simulink model "structure_hifi"  (R2026b)
settings: Solver=VariableStepAuto
undefined symbols (not defined in the file or in its folder): DiscIntNeverNeededParam, P, Ts
settings Model: Creator=aomar  LastModifiedBy=aomar

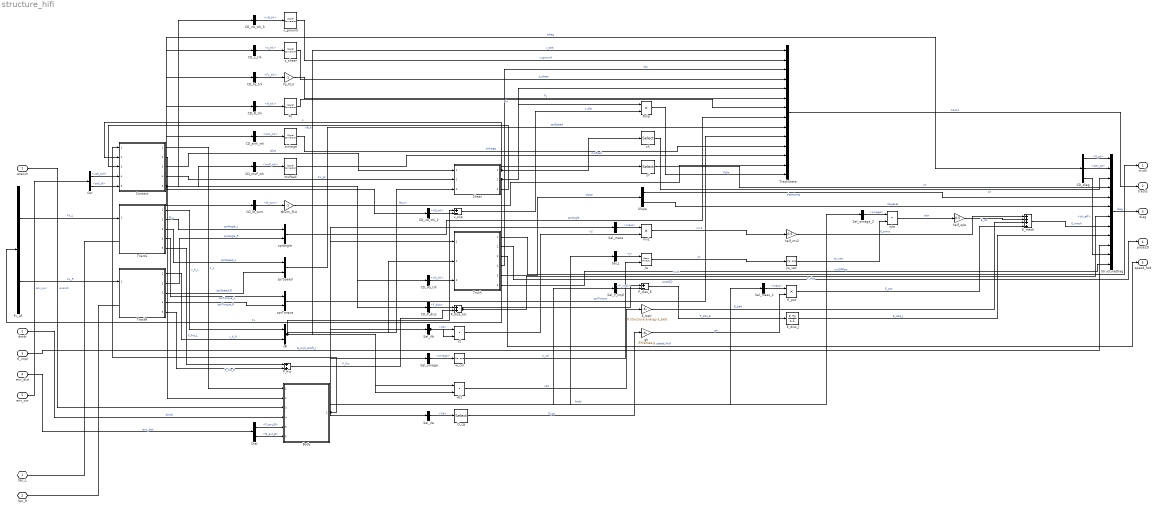
== system structure_hifi ==
  wrench : Inport
  dmdt : Inport  Port=2
  E_impl : Inport  Port=3
  env_dist : Inport  Port=4  OutDataTypeStr=Bus: Bus_EnvDisturbance
  env_ovr : Inport  Port=5  OutDataTypeStr=Bus: Bus_EnvOverride
  Body : Subsystem  ReferencedSubsystem=structure_body6dof
  CD_Fy_trk : BusSelector  OutputSignals=Fy_trk
  CD_M_turn : BusSelector  OutputSignals=M_turn
  CD_N_trk : BusSelector  OutputSignals=N_trk
  CD_P_diss : BusSelector  OutputSignals=P_diss
  CD_diag : BusSelector  OutputSignals=N_pt,pen_pt,chi_eff
  CD_muP_trk : BusSelector  OutputSignals=muP_trk
  CD_s_trk : BusSelector  OutputSignals=s_trk
  CD_sink_trk : BusSelector  OutputSignals=sink_trk
  CD_vG_trk : BusSelector  OutputSignals=vG_trk
  CD_vG_trk_2 : BusSelector  OutputSignals=vG_trk
  CD_vG_trk_3 : BusSelector  OutputSignals=vG_trk
  Contact : Subsystem  ReferencedSubsystem=structure_contact
  D_cg : Selector  InputPortWidth=3  IndexOptions=Index vector (dialog)  Indices=3  OutputSizes=1
  Dist : BusSelector  OutputSignals=F_ext_B,M_ext_B
  E_belt : Gain  Gain=P.structure.energy.k_belt
  E_diss_J : DiscreteIntegrator  gainval=1  SampleTime=Ts.base  ICPrevOutput=DiscIntNeverNeededParam  ICPrevScaledInput=DiscIntNeverNeededParam
  E_mech : Sum  Inputs=++++
  E_pot : Product  Inputs=**
  Fn : SignalConversion  OverrideOpt=off
  Fx_LR : Demux  Outputs=2
  Fy_FLU : Gain  Gain=-1
  Jw : Product  Inputs=**  Multiplication=Matrix(*)
  Jw_vec : Reshape
  Mturn_FLU : Gain  Gain=-1
  Ovr : BusSelector  OutputSignals=use_soil,soil_id
  P_diss_E : Sum  Inputs=+-
  P_diss_tot : Sum
  P_fric : Sum
  Pslip : Product  Inputs=**
  Sel_J : BusSelector  OutputSignals=J
  Sel_P_impl : BusSelector  OutputSignals=P_impl
  Sel_Vb : BusSelector  OutputSignals=Vb
  Sel_Xe : BusSelector  OutputSignals=Xe
  Sel_mass : BusSelector  OutputSignals=mass
  Sel_mass_2 : BusSelector  OutputSignals=mass
  Sel_omega : BusSelector  OutputSignals=omega
  Sel_omega_2 : BusSelector  OutputSignals=omega
  Shear : Subsystem  ReferencedSubsystem=structure_track_shear
  Slope : Demux  Outputs=2
  StructureDiag : BusCreator  Inputs=12  OutDataTypeStr=Bus: Bus_StructureDiag  NonVirtualBus=on
  TrackL : Subsystem  ReferencedSubsystem=structure_track_side  side=1 left
  TrackR : Subsystem  ReferencedSubsystem=structure_track_side  side=2 right
  TrackState : BusCreator  Inputs=14  OutDataTypeStr=Bus: Bus_TrackState  NonVirtualBus=on
  Truth : Subsystem  ReferencedSubsystem=structure_truth
  gh : Gain  Gain=-P.frames.g
  half_mv2 : Gain  Gain=0.5
  half_wJw : Gain  Gain=0.5
  muPeak : SignalConversion  OverrideOpt=off
  mv2 : Product  Inputs=**
  sX : Selector  InputPortWidth=4*P.structure.track.Nc  IndexOptions=Index vector (dialog)  Indices=1:2*P.structure.track.Nc  OutputSizes=1
  sY : Selector  InputPortWidth=4*P.structure.track.Nc  IndexOptions=Index vector (dialog)  Indices=2*P.structure.track.Nc+1:4*P.structure.track.Nc  OutputSizes=1
  s_shear : SignalConversion  OverrideOpt=off
  sinkage : SignalConversion  OverrideOpt=off
  sprAngle : Mux  Inputs=2
  sprSpeed : Mux  Inputs=2
  sprTorque : Mux  Inputs=2
  v2 : DotProduct  OutDataTypeStr=Inherit: Inherit via internal rule
  vB : Mux  Inputs=2
  v_ground : SignalConversion  OverrideOpt=off
  v_slip : Sum  Inputs=+-
  vb2 : DotProduct  OutDataTypeStr=Inherit: Inherit via internal rule
  wJw : DotProduct  OutDataTypeStr=Inherit: Inherit via internal rule
  w_col : Reshape  OutputDimensionality=Column vector (2-D)
  Spr_L : PMIOPort  Side=Left  ConnectionType=Connection: foundation.mechanical.rotational.rotational
  Spr_R : PMIOPort  Port=2  Side=Left  ConnectionType=Connection: foundation.mechanical.rotational.rotational
  truth : Outport  OutDataTypeStr=Bus: Bus_TruthState
  tracks : Outport  Port=2  OutDataTypeStr=Bus: Bus_TrackState
  diag : Outport  Port=3  OutDataTypeStr=Bus: Bus_StructureDiag
  pose2D : Outport  Port=4
  speed_fwd : Outport  Port=5
  wires:
  Fx_LR/1 -> TrackL/1  "Fx_L"
  Fx_LR/2 -> TrackR/1  "Fx_R"
  wrench/1 -> Body/3  "wrench"
  dmdt/1 -> Body/4  "dmdt"
  E_impl/1 -> StructureDiag/10  "E_impl_shaft_J"
  env_dist/1 -> Dist/1  "env_dist"
  env_ovr/1 -> Ovr/1  "env_ovr"
  Ovr/1 -> Contact/4  "<use_soil>"
  Ovr/2 -> Contact/5  "<soil_id>"
  Contact/1 -> Body/1  "F_c"
  Contact/2 -> Body/2  "M_c"
  Contact/3 -> Shear/1  "sDot"
  Contact/4 -> Shear/2  "Fx_pt"
  Contact/5 -> CD_vG_trk_3/1, CD_s_trk/1, CD_P_diss/1, CD_Fy_trk/1, CD_vG_trk/1, CD_N_trk/1, CD_sink_trk/1, CD_vG_trk_2/1, CD_muP_trk/1, CD_M_turn/1, CD_diag/1  "cdiag"
  TrackL/1 -> vB/1  "v_b_L"
  TrackL/2 -> sprAngle/1  "sprAngle_L"
  TrackL/3 -> sprSpeed/1  "sprSpeed_L"
  TrackL/4 -> sprTorque/1  "sprTorque_L"
  TrackL/5 -> P_fric/1  "P_fric_L"
  TrackR/1 -> vB/2  "v_b_R"
  TrackR/2 -> sprAngle/2  "sprAngle_R"
  TrackR/3 -> sprSpeed/2  "sprSpeed_R"
  TrackR/4 -> sprTorque/2  "sprTorque_R"
  TrackR/5 -> P_fric/2  "P_fric_R"
  CD_vG_trk_3/1 -> v_ground/1  "<vG_trk>"
  CD_s_trk/1 -> s_shear/1  "<s_trk>"
  CD_Fy_trk/1 -> Fy_FLU/1  "<Fy_trk>"
  CD_N_trk/1 -> Fn/1  "<N_trk>"
  CD_sink_trk/1 -> sinkage/1  "<sink_trk>"
  CD_muP_trk/1 -> muPeak/1  "<muP_trk>"
  CD_M_turn/1 -> Mturn_FLU/1  "<M_turn>"
  Dist/1 -> Body/5  "<F_ext_B>"
  Dist/2 -> Body/6  "<M_ext_B>"
  sprAngle/1 -> TrackState/8  "sprAngle"
  sprSpeed/1 -> TrackState/9  "sprSpeed"
  sprTorque/1 -> TrackState/10  "sprTorque"
  vB/1 -> TrackState/1, Shear/3, v_slip/1, Truth/2, vb2/2, vb2/1  "v_belt"
  P_fric/1 -> P_diss_tot/2  "P_fric"
  Fy_FLU/1 -> TrackState/6  "Fy"
  Mturn_FLU/1 -> TrackState/13  "Mturn"
  v_ground/1 -> TrackState/2  "v_ground"
  s_shear/1 -> TrackState/4  "s_shear"
  Fn/1 -> TrackState/7  "Fn"
  sinkage/1 -> TrackState/11  "sinkage"
  muPeak/1 -> TrackState/12  "muPeak"
  Body/1 -> Contact/1, Sel_omega_2/1, Sel_mass/1, Truth/1, Sel_J/1, Sel_P_impl/1, Sel_mass_2/1, Sel_Vb/1, Sel_omega/1, Sel_Xe/1  "body"
  CD_vG_trk_2/1 -> v_slip/2  "<vG_trk>"
  CD_vG_trk/1 -> Truth/3  "<vG_trk>"
  CD_P_diss/1 -> P_diss_tot/1  "<P_diss>"
  Sel_Vb/1 -> v2/2, v2/1  "<Vb>"
  Sel_omega/1 -> w_col/1  "<omega>"
  Sel_Xe/1 -> D_cg/1  "<Xe>"
  v_slip/1 -> Pslip/2  "v_slip"
  P_diss_tot/1 -> StructureDiag/7, P_diss_E/1  "P_diss"
  v2/1 -> mv2/2  "v2"
  w_col/1 -> Jw/2  "w_col"
  vb2/1 -> E_belt/1  "vb2"
  D_cg/1 -> gh/1  "D_cg"
  Shear/1 -> sX/1, Contact/2, sY/1  "s"
  Shear/2 -> TrackState/5, Pslip/1, Fx_LR/1  "Fx"
  Shear/3 -> Contact/3  "vB_d"
  Truth/1 -> truth/1  "truth"
  Truth/2 -> pose2D/1  "pose2D"
  Truth/3 -> speed_fwd/1  "speed_fwd"
  Truth/4 -> TrackState/3  "slip"
  Truth/5 -> Slope/1  "slope"
  Truth/6 -> StructureDiag/12  "outOfMap"
  Sel_mass/1 -> mv2/1  "<mass>"
  Sel_J/1 -> Jw/1  "<J>"
  Sel_P_impl/1 -> P_diss_E/2  "<P_impl>"
  Slope/1 -> StructureDiag/5  "slopeLong"
  Slope/2 -> StructureDiag/6  "slopeLat"
  P_diss_E/1 -> E_diss_J/1  "P_diss_E"
  Pslip/1 -> TrackState/14  "Pslip"
  mv2/1 -> half_mv2/1  "mv2"
  Jw/1 -> Jw_vec/1  "Jw"
  E_belt/1 -> E_mech/3  "E_belt"
  gh/1 -> E_pot/2  "gh"
  sX/1 -> StructureDiag/3  "sX"
  sY/1 -> StructureDiag/4  "sY"
  Sel_mass_2/1 -> E_pot/1  "<mass>"
  TrackState/1 -> tracks/1  "tracks"
  half_mv2/1 -> E_mech/1  "E_trans"
  Jw_vec/1 -> wJw/2  "Jw_vec"
  E_pot/1 -> E_mech/4  "E_pot"
  E_diss_J/1 -> StructureDiag/9  "E_diss_J"
  Sel_omega_2/1 -> wJw/1  "<omega>"
  wJw/1 -> half_wJw/1  "wJw"
  half_wJw/1 -> E_mech/2  "E_rot"
  E_mech/1 -> StructureDiag/8  "E_mech"
  CD_diag/1 -> StructureDiag/1  "<N_pt>"
  CD_diag/2 -> StructureDiag/2  "<pen_pt>"
  CD_diag/3 -> StructureDiag/11  "<chi_eff>"
  StructureDiag/1 -> diag/1  "diag"
  connections:
  TrackL/LConn1 -- Spr_L/RConn1
  TrackR/LConn1 -- Spr_R/RConn1
